simulink model "Lab2_VM_Task_5678"  (R2025a)
settings: Solver=VariableStepAuto  StartTime=0.0  StopTime=10.0  RelTol=1e-3
undefined symbols (not defined in the file or in its folder): Angular, Linear
libraries: robotlib x4
settings Model: Creator=Sina  LastModifiedBy=david
settings SolverCC: AlgebraicLoopSolver=TrustRegion
settings DataIOCC: ReturnWorkspaceOutputs=off
settings DebuggingCC: UnconnectedInputMsg=warning  UnconnectedOutputMsg=warning  UnconnectedLineMsg=warning  ArithmeticOperatorsInVariantConditions=warning
settings ModelReferenceCC: EnableRefExpFcnMdlSchedulingChecks=on
settings SFSimCC: SimUseLocalCustomCode=off  CustomCodeUndefinedFunction=UseInterfaceOnly
settings RTWCC: RTWUseLocalCustomCode=off  GPUComputeCapability=3.5

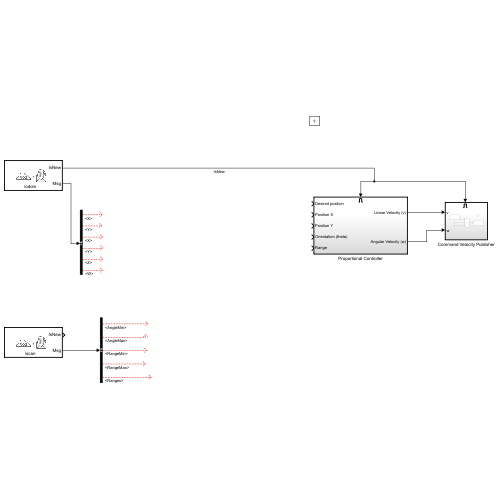
[thumbnail: Simulink's stored preview of the top-level diagram]
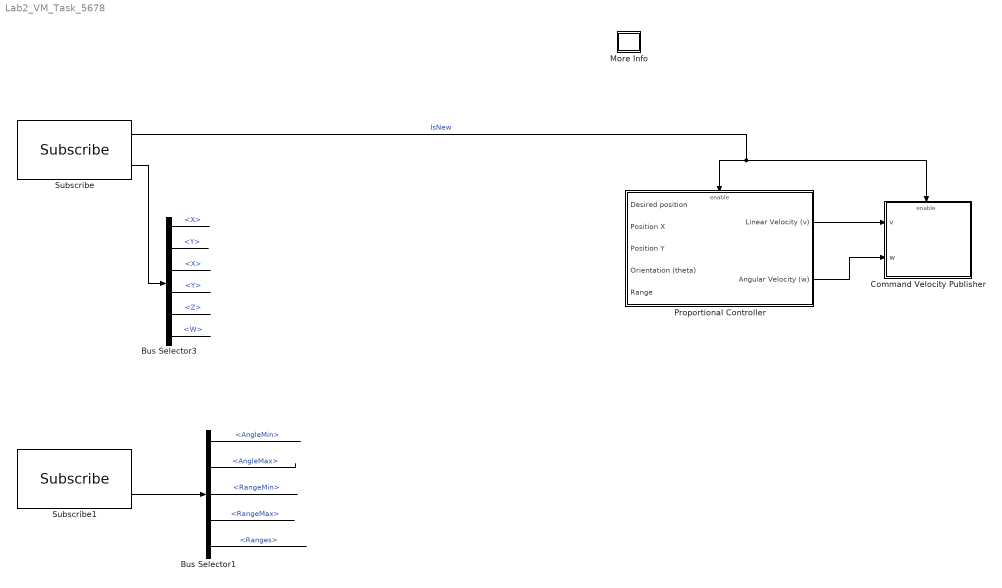
== system Lab2_VM_Task_5678 ==
  Bus Selector1 : BusSelector  OutputSignals=AngleMin,AngleMax,RangeMin,RangeMax,Ranges
  Bus Selector3 : BusSelector  OutputSignals=Pose.Pose.Position.X,Pose.Pose.Position.Y,Pose.Pose.Orientation.X,Pose.Pose.Orientation.Y,Pose.Pose.Orientation.Z,Pose.Pose.Orientation.W
  Command Velocity Publisher : Subsystem
  More Info : Subsystem
      settings: OpenFcn=showdemo(bdroot(gcb))
      mask Display: disp('?')
  Proportional Controller : Subsystem
  Subscribe : robotlib/Subscribe  topicSource=Select from ROS network  topic=/odom  messageType=nav_msgs/Odometry  SampleTime=-1  legacyBusStruct=off  messageQueueLength=51
  Subscribe1 : robotlib/Subscribe  topicSource=Select from ROS network  topic=/scan  messageType=sensor_msgs/LaserScan  SampleTime=-1  legacyBusStruct=off  messageQueueLength=51
  wires:
  Bus Selector3/2 -> ?  "<Y>"
  Bus Selector3/1 -> ?  "<X>"
  Proportional Controller/2(Angular Velocity (w)) -> Command Velocity Publisher/2(w)
  Subscribe/1 -> Command Velocity Publisher/Enable, Proportional Controller/Enable  "IsNew"
  Bus Selector3/5 -> ?  "<Z>"
  Proportional Controller/1(Linear Velocity (v)) -> Command Velocity Publisher/1(v)
  Bus Selector3/3 -> ?  "<X>"
  Subscribe/2 -> Bus Selector3/1
  Bus Selector3/4 -> ?  "<Y>"
  Bus Selector3/6 -> ?  "<W>"
  Bus Selector1/3 -> ?  "<RangeMin>"
  Bus Selector1/4 -> ?  "<RangeMax>"
  Bus Selector1/2 -> ?  "<AngleMax>"
  Bus Selector1/5 -> ?  "<Ranges>"
  Subscribe1/2 -> Bus Selector1/1
  Bus Selector1/1 -> ?  "<AngleMin>"

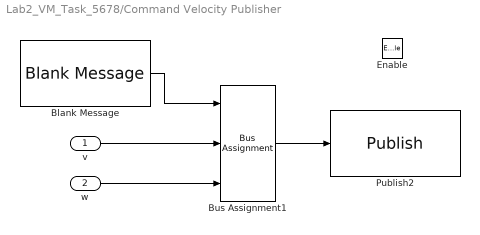
== system Lab2_VM_Task_5678/Command Velocity Publisher ==
  v : Inport
  w : Inport  Port=2
  Enable : EnablePort
  Blank Message : robotlib/Blank Message  SourceLibraryInfo=This block requires Robotics System Toolbox  messageType=geometry_msgs/Twist  SampleTime=inf
  Bus Assignment1 : BusAssignment  DialogController=Simulink.DDGSource_BusAssignment  AssignedSignals=Linear.X,Angular.Z
  Publish2 : robotlib/Publish  SourceLibraryInfo=This block requires Robotics System Toolbox  topicSource=Select from ROS network  topic=/cmd_vel  messageType=geometry_msgs/Twist  messageQueueLength=105
  wires:
  Bus Assignment1/1 -> Publish2/1
  Blank Message/1 -> Bus Assignment1/1
  v/1 -> Bus Assignment1/2
  w/1 -> Bus Assignment1/3

== system Lab2_VM_Task_5678/More Info ==

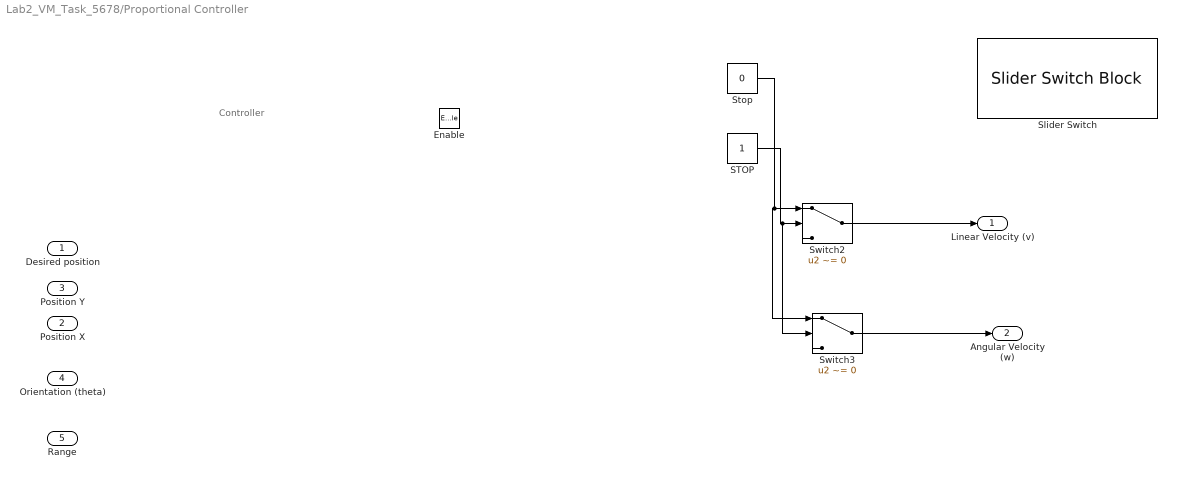
== system Lab2_VM_Task_5678/Proportional Controller ==
  note: Controller
  Desired position : Inport
  Position X : Inport  Port=2
  Position Y : Inport  Port=3
  Orientation (theta) : Inport  Port=4
  Range : Inport  Port=5
  Enable : EnablePort
  "STOP " : Constant
  Slider Switch : SliderSwitchBlock
  Stop : Constant  Value=0
  Switch2 : Switch  Criteria=u2 ~= 0  SaturateOnIntegerOverflow=off  InputSameDT=off
  Switch3 : Switch  Criteria=u2 ~= 0  SaturateOnIntegerOverflow=off  InputSameDT=off
  Linear Velocity (v) : Outport  VectorParamsAs1DForOutWhenUnconnected=off
  Angular Velocity (w) : Outport  Port=2  VectorParamsAs1DForOutWhenUnconnected=off
  wires:
  Stop/1 -> Switch3/1, Switch2/1
  "STOP "/1 -> Switch3/2, Switch2/2
  Switch2/1 -> Linear Velocity (v)/1
  Switch3/1 -> Angular Velocity (w)/1
